simulink model "G22_Simulink"  (R2026a)
settings: Solver=VariableStepAuto  StopTime=1000
libraries: cstblocks_lti x1
settings Model: Creator=nelis  LastModifiedBy=nelis

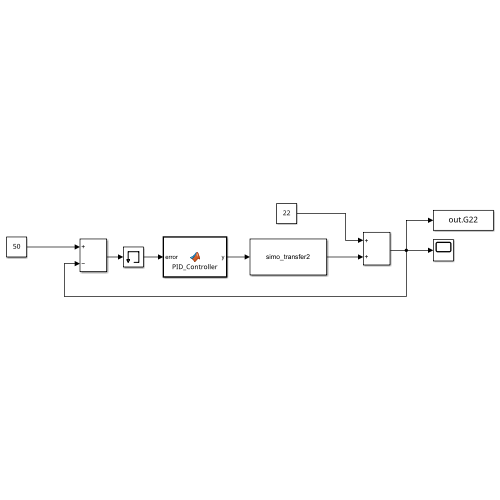
[thumbnail: Simulink's stored preview of the top-level diagram]
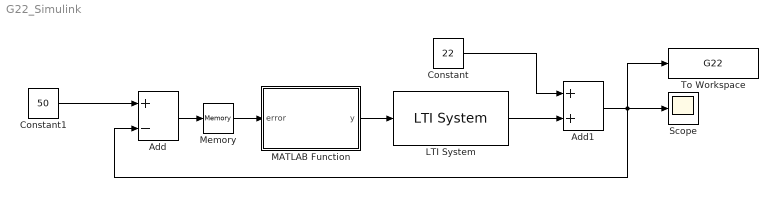
== system G22_Simulink ==
  Add : Sum  Inputs=+-
  Add1 : Sum
  Constant : Constant  Value=22
  Constant1 : Constant  Value=50
  LTI System : cstblocks_lti/LTI System  sys=simo_transfer2  IC=[]  PadeOrder=1
      settings: LibrarySourceBlock=cstblocks/LTI System
  MATLAB Function : MATLAB Function  TreatAsAtomicUnit=on  SystemSampleTime=0.005
  Memory : Memory
  Scope : Scope
      settings: ActiveDisplayYMinimum=20.108688006545385  ActiveDisplayYMaximum=39.021807941091531
  To Workspace : ToWorkspace  VariableName=G22  SaveFormat=Timeseries  SampleTime=-1
  wires:
  Add/1 -> Memory/1
  Constant1/1 -> Add/1
  Constant/1 -> Add1/1
  Add1/1 -> To Workspace/1, Scope/1, Add/2
  Memory/1 -> MATLAB Function/1(error)
  MATLAB Function/1(y) -> LTI System/1
  LTI System/1 -> Add1/2

== matlab function G22_Simulink/MATLAB Function ==
  data: y output; error input
function y =  PID_Controller(error)
    persistent prev_error;
    persistent integral;
    dt = 0.005;

    D = 1.90571;
    P = 0.2329;
    I = 0.004226;

    if isempty(prev_error)
        prev_error = error;
    end

    if isempty(integral)
        integral = 0;
    end

    next_integral = integral + error * dt;
    derivative = (error - prev_error)/dt;

    pid_out = P*error + I*next_integral + D*derivative;

    if pid_out >= 3.3
        pid_out = 3.3;
        if error < 0
            integral = next_integral;
        end

    elseif pid_out < 0
        pid_out = 0;
        if error > 0
            integral = next_integral;
        end
    else
        integral = next_integral;
    end

    prev_error = error;

y = pid_out;
